simulink model "FCSMPC_new"  (R2026a)
settings: Solver=FixedStepDiscrete  StopTime=inf  FixedStep=SimulinkTs
PreLoadFcn:
  | % Verzeichnis des Modells zum MATLAB-Pfad hinzufügen
  | modelDir = fileparts(get_param(bdroot, 'FileName'));
  | addpath(modelDir);
  | 
  | % Nur der Dateiname – kein Pfad!
  | set_param(bdroot, 'DataDictionary', 'FOC_params.sldd');
model workspace (MAT data in the model file):
  Np : Simulink.Parameter (value not decoded)
undefined symbols (not defined in the file or in its folder): dspblkCoreblockFVToolHelper, FCS, Filter, FOC, FOC_Control_Current_KIid, FOC_Control_Current_KIiq, FOC_Control_Current_KPid, FOC_Control_Current_KPiq, FOC_Control_Current_Krd, FOC_Control_Current_Krq, FOC_Control_Current_TclCur, FOC_Control_Current_Tnd, FOC_Control_Current_Tnq, FOC_Control_InverterVdc_V, FOC_Control_MotorImax_A, FOC_Control_MTPA_MTPV_nT_id_grid, FOC_Control_MTPA_MTPV_nT_iq_grid, FOC_Control_MTPA_MTPV_T_vec, FOC_Control_MTPA_MTPV_w_vec, FOC_Control_OpenLoop_Id_Ref_A, FOC_Control_OpenLoop_Iq_Ref_A, FOC_Control_OpenLoop_Ud_OpenLoop_V, FOC_Control_OpenLoop_Uq_OpenLoop_V, FOC_Control_RF_omegamech_rad_s, FOC_Control_RF_RateCurrent_A, FOC_Control_RF_RateTrq_Nm, FOC_Control_theta_mechOffsetFix, FOC_Control_theta_mechOffsetTime, FOC_Control_TorqueRef_Nm, FOC_Control_Umax_V, FOC_Flag_ClosedLoopControl, FOC_Flag_ControlStrategy, FOC_Flag_PWMEnable, FOC_Flag_ResetControl, FOC_Flag_TorqueControl, FOC_LUT_DQLimiter_DQ_LUTScaling, FOC_PWM_AZSPWMMethod, FOC_PWM_HybridMode, FOC_PWM_LB1, FOC_PWM_LB2, FOC_PWM_PWMManuel, FOC_PWM_RSPWMMethod, FOC_PWM_UB1, FOC_PWM_UB2, FOC_SampleTime_TsCur, gcbh, Plant, SimulinkTs
libraries: hdlsllib x2, autolibfluxpmsm x1, simulink x1
(part 2 of 2)

== matlab function FCSMPC_new/FCS_MPC/SDA_Solve/SDA Solve/Assembly_QP ==
  data: Ad input; Bd input; fd input; H output size=[3*Np 3*Np]; Gamma input; U_unc output size=[3*Np 1]; Phi input; Apow input; Lambdafsw_Ssquare input; Lambdafsw_SE input; Bs_TI input; Iabc input; idiq_ref input; Sin_Cos_Theta input size=[2 1]; Sin_Cos_Theta_Delayed input; wel input; Ts input; U_applied input; regularization input; controllerDelay input; iabcPredictedPrevious input; predictionValid input; iabcCompensated output; deltaIabcBase output; deltaIabcSwitch output; predictionError output size=[3 1]; e_dq output size=[2 1]
function [H, U_unc, iabcCompensated, ...
    deltaIabcBase, deltaIabcSwitch, predictionError, e_dq] = ...
    Assembly_QP(Ad, Bd, fd, Gamma, Phi, Apow, ...
    Lambdafsw_Ssquare, Lambdafsw_SE, Bs_TI, ...
    Iabc, idiq_ref, Sin_Cos_Theta, Sin_Cos_Theta_Delayed, ...
    wel, Ts, U_applied, ...
    regularization, controllerDelay, ...
    iabcPredictedPrevious, predictionValid)
%ASSEMBLY_QP Independent QP-assembly MATLAB Function module.
% Sin_Cos_Theta = [sin(theta_el); cos(theta_el)] at the current instant.
% Sin_Cos_Theta_Delayed is the same signal delayed by one SDA period.
% U_applied is a fixed 6x1 vector delayed by one SDA period and contains the
% two switching vectors that were physically applied during the measurement
% delay, ordered oldest first:
%   U_applied = [Uapply(k-1); UapplySecond(k-1)].
% The last applied switching state is therefore U_applied(4:6).
% With controllerDelay = 40 us and Ts = 20 us, both history steps are used
% to propagate the delayed current measurement to the current instant.
% iabcPredictedPrevious is supplied by a model-level Unit Delay block.

Np = 5;
ns = 3;
nS = ns*Np;

% The surrounding FOC model may provide fixed-point fi signals. This QP
% stage uses matrix factorizations and linear solves, so perform all of its
% numerical work consistently in double precision. Mixing a run-time fi
% value with a non-fi matrix in mtimes is not supported by MATLAB Coder.
Ad = double(Ad);
Bd = double(Bd);
fd = double(fd);
Gamma = double(Gamma);
Phi = double(Phi);
Apow = double(Apow);
Lambdafsw_Ssquare = double(Lambdafsw_Ssquare);
Lambdafsw_SE = double(Lambdafsw_SE);
Bs_TI = double(Bs_TI);
Iabc = double(Iabc);
idiq_ref = double(idiq_ref);
Sin_Cos_Theta = double(Sin_Cos_Theta);
Sin_Cos_Theta_Delayed = double(Sin_Cos_Theta_Delayed);
wel = double(wel);
Ts = double(Ts);
U_applied = double(U_applied);
regularization = double(regularization);
controllerDelay = double(controllerDelay);
iabcPredictedPrevious = double(iabcPredictedPrevious);

sinTheta = Sin_Cos_Theta(1);
cosTheta = Sin_Cos_Theta(2);
thetaCurrent = atan2(sinTheta,cosTheta);
thetaDelayed = atan2( ...
    Sin_Cos_Theta_Delayed(1),Sin_Cos_Theta_Delayed(2));
Talpha_beta = [2/3, -1/3, -1/3; ...
               0, 1/sqrt(3), -1/sqrt(3)];

uprev = U_applied(4:6);

% Reconstruct the present current from the delayed measurement by replaying
% the switching vectors that were physically applied during that delay.
% The fixed upper loop bound keeps dimensions/code generation deterministic.
delaySteps = 0;
if predictionValid
    delaySteps = min(2,max(0,round(controllerDelay/Ts)));
end
iabcCompensated = Iabc;
thetaHistoryStart = thetaCurrent;
if delaySteps == 2
    % The supplied delayed angle is one complete SDA period (2*Ts) old.
    thetaHistoryStart = thetaDelayed;
elseif delaySteps == 1
    % A one-step delay corresponds to the second half of the previous SDA
    % period. The supplied delayed angle is 2*Ts old, so use the current
    % angle and constant-speed assumption to obtain the angle Ts ago.
    thetaHistoryStart = thetaCurrent-wel*Ts;
end
for historyStep = 1:2
    if historyStep <= delaySteps
        thetaHistory = thetaHistoryStart+(historyStep-1)*wel*Ts;
        [deltaBaseHistory,deltaSwitchHistory] = abc_current_increment( ...
            iabcCompensated,thetaHistory,Ad,Bd,fd,Bs_TI,wel,Ts);
        % For two delay steps replay [U1(k-1), U2(k-1)]. For one delay
        % step replay only the most recently applied U2(k-1).
        historySlot = 2-delaySteps+historyStep;
        historyIndices = (historySlot-1)*ns+(1:ns);
        sHistory = U_applied(historyIndices);
        iabcCompensated = iabcCompensated+ ...
            deltaBaseHistory+deltaSwitchHistory*sHistory;
    end
end

% Build the optimization and future-prediction model from the reconstructed
% current state at the current electrical angle.
[deltaIabcBase,deltaIabcSwitch,idiq_fb,Rpark,Bs] = ...
    abc_current_increment( ...
        iabcCompensated,thetaCurrent,Ad,Bd,fd,Bs_TI,wel,Ts);

Upsilon = zeros(2*Np,ns*Np);
for row = 1:Np
    rows = (row-1)*2 + (1:2);
    for col = 1:row
        cols = (col-1)*ns + (1:ns);
        Upsilon(rows,cols) = ...
            Apow((row-col)*2 + (1:2),:)*Bd*Bs;
    end
end

if predictionValid
    predictionError = iabcCompensated-iabcPredictedPrevious;
else
    predictionError = zeros(3,1);
end
e_dq = Rpark*(Talpha_beta*predictionError);

Yref = repmat(idiq_ref,Np,1);
r = Yref-Gamma*idiq_fb-Phi;
W = Upsilon.'*Upsilon + Lambdafsw_Ssquare;
Theta = -Upsilon.'*r-Lambdafsw_SE*uprev;
W = 0.5*(W+W.');
scaleH = max(1,norm(W,'fro'));
W = W+regularization*scaleH*eye(nS);
U_unc = W\(-Theta);

Jx = fliplr(eye(nS));
[Rt,cholFlag] = chol(Jx*W*Jx);
if cholFlag ~= 0
    error('H is not positive definite. Increase lambda_sw or regularization.');
end
H = Jx*Rt*Jx;
end

function [deltaBase,deltaSwitch,idiqState,Rpark,Bs] = ...
    abc_current_increment( ...
        iabcState,thetaEl,Ad,Bd,fd,Bs_TI,wel,Ts)
% One discrete PMSM current step in abc coordinates at thetaEl.
cosTheta = cos(thetaEl);
sinTheta = sin(thetaEl);
Rpark = [cosTheta, sinTheta; -sinTheta, cosTheta];
Talpha_beta = [2/3, -1/3, -1/3; ...
               0, 1/sqrt(3), -1/sqrt(3)];
TinvClarke = [1.0, 0.0; ...
             -0.5, sqrt(3)/2; ...
             -0.5, -sqrt(3)/2];
Jrot = [0 -1; 1 0];

idiqState = Rpark*(Talpha_beta*iabcState);
Bs = Rpark*Bs_TI;
Tdq2abc = TinvClarke*Rpark.';
deltaIdqBase = (Ad-eye(2))*idiqState+fd;
deltaBase = Tdq2abc* ...
    (deltaIdqBase+Jrot*idiqState*(wel*Ts));
deltaSwitch = Tdq2abc*Bd*Bs;
end

== matlab function FCSMPC_new/FCS_MPC/SDA_Solve/SDA Solve/SDA_Solve ==
  data: Jopt output size=[1 1]; nodes output size=[1 1]; optimal output size=[1 1]; H input size=[15 15]; U_unc input size=[15 1]; NmaxNod input size=[1 1]; Uopt output size=[3*Np 1]; Uapply output size=[3]; UoptPrev input size=[15 1]; iabcCompensated input size=[3 1]; deltaIabcBase input size=[3 1]; deltaIabcSwitch input size=[3 3]; lambdaZero input size=[1 1]; lambdaDeadtime input size=[1 1]; deadtime_ratio input size=[1 1]; currentEpsMargin input size=[1 1]; UapplySecond output size=[3 1]; leafNodes output size=[1 1]; bestCMVCost output size=[1 1]; cmvMetricRatio output size=[1 1]; switchCountApplied output size=[1 1]; debug_lower output size=[3 1]; debug_upper output size=[3 1]; iabcPredictedNext output size=[3 1]; Jround output size=[1 1]; Jshift output size=[1 1]; predictionValidNext output boolean size=[1 1]
function [Jopt, nodes, optimal, Uopt, Uapply, UapplySecond, ...
    leafNodes, bestCMVCost, cmvMetricRatio, switchCountApplied, ...
    debug_lower, debug_upper, iabcPredictedNext, ...
    Jround, Jshift, predictionValidNext] = ...
    SDA_Solve(H, U_unc, NmaxNod, UoptPrev, ...
    iabcCompensated, deltaIabcBase, deltaIabcSwitch, ...
    lambdaZero, lambdaDeadtime, deadtime_ratio, currentEpsMargin)
%SDA_SOLVE Independent double-vector SDA MATLAB Function module.
% The first five ports follow FCSMPC_IdealSDA. Feed Uopt back to UoptPrev
% through a Unit Delay initialized with zeros(15,1). Uapply and
% UapplySecond are applied successively for half an external period each.

Np = 5;
ns = 3;
nS = ns*Np;

z = H*U_unc;
s_prev = UoptPrev(4:6);
deadtimeRatio = deadtime_ratio;

Uround = min(max(round(U_unc),0.0),1.0);
Ushift = zeros(nS,1);
Ushift(1:nS-ns) = UoptPrev(ns+1:nS);
Ushift(nS-ns+1:nS) = UoptPrev(nS-ns+1:nS);
Jround = norm(H*(Uround-U_unc),2)^2;
Jshift = norm(H*(Ushift-U_unc),2)^2;
if Jshift < Jround
    U_ini = Ushift;
else
    U_ini = Uround;
end

bestCMVCost = sequence_cmv_cost_predicted( ...
    U_ini,s_prev,iabcCompensated,Np,ns, ...
    deltaIabcBase,deltaIabcSwitch,lambdaZero,lambdaDeadtime, ...
    deadtimeRatio,currentEpsMargin);
bestMetric = norm(H*(U_ini-U_unc),2)^2+bestCMVCost;
bestU = U_ini;

Uwork = zeros(nS,1);
candidatePosition = ones(nS,1);
metricStack = zeros(nS+1,1);
cmvMetricStack = zeros(nS+1,1);
iabcPrediction = zeros(3,Np+1);
iabcPrediction(:,1) = iabcCompensated;
nodes = 0;
leafNodes = 0;
optimal = true;
i = 1;

while i >= 1
    if candidatePosition(i) > 2
        candidatePosition(i) = 1;
        i = i-1;
        continue;
    end
    head = 0.0;
    if i > 1
        head = H(i,1:i-1)*Uwork(1:i-1);
    end
    center = (z(i)-head)/H(i,i);
    if center <= 0.5
        firstCandidate = 0.0;
    else
        firstCandidate = 1.0;
    end
    if candidatePosition(i) == 1
        candidate = firstCandidate;
    else
        candidate = 1.0-firstCandidate;
    end
    candidatePosition(i) = candidatePosition(i)+1;
    Uwork(i) = candidate;
    nodes = nodes+1;
    if NmaxNod > 0 && nodes > NmaxNod
        optimal = false;
        break;
    end

    residual = z(i)-head-H(i,i)*candidate;
    metricNew = metricStack(i)+residual*residual;
    cmvMetricNew = cmvMetricStack(i);
    if mod(i,ns) == 0
        predictionStep = i/ns;
        blockStart = i-ns+1;
        sCurrent = Uwork(blockStart:i);
        if predictionStep == 1
            sPrevious = s_prev;
        else
            sPrevious = Uwork(blockStart-ns:blockStart-1);
        end
        iabcBeforeSwitch = iabcPrediction(:,predictionStep);
        [deltaStep,deltaDead] = deadtime_corrected_current_step( ...
            sPrevious,sCurrent,iabcBeforeSwitch, ...
            deltaIabcBase,deltaIabcSwitch,deadtimeRatio,currentEpsMargin);
        cmvIncrement = cmv_cost( ...
            sPrevious,sCurrent,iabcBeforeSwitch,deltaDead, ...
            lambdaZero,lambdaDeadtime,currentEpsMargin);
        metricNew = metricNew+cmvIncrement;
        cmvMetricNew = cmvMetricNew+cmvIncrement;
        iabcPrediction(:,predictionStep+1) = iabcBeforeSwitch+deltaStep;
    end
    if metricNew > bestMetric
        continue;
    end
    if i == nS
        leafNodes = leafNodes+1;
        if metricNew < bestMetric
            bestMetric = metricNew;
            bestU = Uwork;
            bestCMVCost = cmvMetricNew;
        end
    else
        metricStack(i+1) = metricNew;
        cmvMetricStack(i+1) = cmvMetricNew;
        i = i+1;
        candidatePosition(i) = 1;
    end
end

if isfinite(bestMetric)
    Uopt = bestU;
else
    Uopt = repmat(s_prev,Np,1);
end
Uapply = Uopt(1:3);
UapplySecond = Uopt(4:6);

[deltaFirst,~] = deadtime_corrected_current_step( ...
    s_prev,Uapply,iabcCompensated, ...
    deltaIabcBase,deltaIabcSwitch, ...
    deadtimeRatio,currentEpsMargin);
iabcAfterFirst = iabcCompensated + deltaFirst;

[deltaSecond,~] = deadtime_corrected_current_step( ...
    Uapply,UapplySecond,iabcAfterFirst, ...
    deltaIabcBase,deltaIabcSwitch,deadtimeRatio,currentEpsMargin);
iabcPredictedNext = iabcAfterFirst+deltaSecond;

switchCountApplied = sum(abs(Uapply-s_prev))+ ...
    sum(abs(UapplySecond-Uapply));
Jopt = bestMetric;
if Jopt > eps
    cmvMetricRatio = bestCMVCost/Jopt;
else
    cmvMetricRatio = 0.0;
end
[~,debugDeltaDead] = deadtime_corrected_current_step( ...
    s_prev,Uapply,iabcCompensated,deltaIabcBase,deltaIabcSwitch, ...
    deadtimeRatio,currentEpsMargin);
[~,debug_lower,debug_upper] = cmv_cost( ...
    s_prev,Uapply,iabcCompensated,debugDeltaDead, ...
    lambdaZero,lambdaDeadtime,currentEpsMargin);
predictionValidNext = true;
end

function [deltaStep,deltaDead] = deadtime_corrected_current_step( ...
    sPrevious,sCurrent,iabcBeforeSwitch, ...
    deltaBase,deltaSwitch,deadtimeRatio,currentEps)
sDead = sCurrent;
changed = (sPrevious ~= sCurrent);
signEps = 0.1*currentEps;
for phase = 1:3
    if ~changed(phase)
        continue;
    end
    iPhase = iabcBeforeSwitch(phase);
    if iPhase >= signEps
        sDead(phase) = 0.0;
    elseif iPhase <= -signEps
        sDead(phase) = 1.0;
    else
        sDead(phase) = 0.5*(1.0-iPhase/signEps);
    end
end
sEffective = deadtimeRatio*sDead+(1.0-deadtimeRatio)*sCurrent;
deltaDead = deadtimeRatio*(deltaBase+deltaSwitch*sDead);
deltaStep = deltaBase+deltaSwitch*sEffective;
end

function [penalty,lowerBound,upperBound] = cmv_cost( ...
    sPrevious,sCurrent,iabcBeforeSwitch,deltaDead, ...
    lambdaZero,lambdaDeadtime,currentEpsMargin)
penalty = 0.0;
iabcDeadEnd = iabcBeforeSwitch+deltaDead;
lowerBound = min(iabcBeforeSwitch,iabcDeadEnd)-currentEpsMargin;
upperBound = max(iabcBeforeSwitch,iabcDeadEnd)+currentEpsMargin;
uncertain = (lowerBound <= 0.0) & (upperBound >= 0.0);
if all(sCurrent == 0.0) || all(sCurrent == 1.0)
    penalty = penalty+lambdaZero;
end
changed = (sPrevious ~= sCurrent);
if sum(changed) ~= 2
    return;
end
canBeZero = false(3,1);
canBeOne = false(3,1);
for phase = 1:3
    if ~changed(phase)
        canBeZero(phase) = (sPrevious(phase) == 0.0);
        canBeOne(phase) = (sPrevious(phase) == 1.0);
    elseif uncertain(phase)
        canBeZero(phase) = true;
        canBeOne(phase) = true;
    elseif iabcDeadEnd(phase) > 0.0
        canBeZero(phase) = true;
    else
        canBeOne(phase) = true;
    end
end
if all(canBeZero) || all(canBeOne)
    penalty = penalty+lambdaDeadtime;
end
end

function totalPenalty = sequence_cmv_cost_predicted( ...
    U,s_prev,iabcInitial,Np,ns,deltaBase,deltaSwitch, ...
    lambdaZero,lambdaDeadtime,deadtimeRatio,currentEpsMargin)
totalPenalty = 0.0;
sPrevious = s_prev;
iabcBeforeSwitch = iabcInitial;
for step = 1:Np
    rows = (step-1)*ns+(1:ns);
    sCurrent = U(rows);
    [deltaStep,deltaDead] = deadtime_corrected_current_step( ...
        sPrevious,sCurrent,iabcBeforeSwitch,deltaBase,deltaSwitch, ...
        deadtimeRatio,currentEpsMargin);
    totalPenalty = totalPenalty+cmv_cost( ...
        sPrevious,sCurrent,iabcBeforeSwitch,deltaDead, ...
        lambdaZero,lambdaDeadtime,currentEpsMargin);
    iabcBeforeSwitch = iabcBeforeSwitch+deltaStep;
    sPrevious = sCurrent;
end
end

== stateflow chart FCSMPC_new/FCS_MPC/CurrentRefCalc/Current_RateLimiter/RateLimiter ==
  settings: updateMethod=DISCRETE  sampleTime=FOC.SampleTime.TsSpeed
  state IDLE
  state Rising
    entry:  y =  fi(y_prev +dT * R, 1, 32, 18);
    exit: y_prev = y;
  state Falling
    entry:  y = fi(y_prev+dT * F, 1, 32, 18);
    exit: y_prev = y;
  state Directpassage
    entry:  y = u;
    exit: y_prev = y;
  (default) -> IDLE
  IDLE -> (junction 22)
  (junction 22) -> Rising [order 1] : [(u-y_prev)/dT>=R]
  (junction 22) -> Falling [order 2] : [(u-y_prev)/dT<=F]
  Rising -> (junction 22)
  Falling -> (junction 22)
  Directpassage -> (junction 22)
  (junction 22) -> Directpassage [order 3] : [(u-y_prev)/dT<R && (u-y_prev)/dT>F]
  data: u input fixdt(1,32,18); R input fixdt(1,32,18); F input fixdt(1,32,18); dT constant fixdt(1,32,18) size=1 =FOC.SampleTime.TsSpeed; y output fixdt(1,32,18); y_prev local fixdt(1,32,18) =0

== stateflow chart FCSMPC_new/FCS_MPC/CurrentRefCalc/Current_RateLimiter/RateLimiter1 ==
  settings: updateMethod=DISCRETE  sampleTime=FOC.SampleTime.TsSpeed
  state IDLE
  state Rising
    entry:  y =  fi(y_prev +dT * R, 1, 32, 18);
    exit: y_prev = y;
  state Falling
    entry:  y = fi(y_prev+dT * F, 1, 32, 18);
    exit: y_prev = y;
  state Directpassage
    entry:  y = u;
    exit: y_prev = y;
  (default) -> IDLE
  IDLE -> (junction 22)
  (junction 22) -> Rising [order 1] : [(u-y_prev)/dT>=R]
  (junction 22) -> Falling [order 2] : [(u-y_prev)/dT<=F]
  Rising -> (junction 22)
  Falling -> (junction 22)
  Directpassage -> (junction 22)
  (junction 22) -> Directpassage [order 3] : [(u-y_prev)/dT<R && (u-y_prev)/dT>F]
  data: u input fixdt(1,32,18); R input fixdt(1,32,18); F input fixdt(1,32,18); dT constant fixdt(1,32,18) size=1 =FOC.SampleTime.TsSpeed; y output fixdt(1,32,18); y_prev local fixdt(1,32,18) =0

== stateflow chart FCSMPC_new/FCS_MPC/CurrentRefCalc/RateLimiter ==
  settings: updateMethod=DISCRETE  sampleTime=FOC.SampleTime.TsSpeed
  state IDLE
  state Rising
    entry:  y =  fi(y_prev +dT * R, 1, 32, 18);
    exit: y_prev = y;
  state Falling
    entry:  y = fi(y_prev+dT * F, 1, 32, 18);
    exit: y_prev = y;
  state Directpassage
    entry:  y = u;
    exit: y_prev = y;
  (default) -> IDLE
  IDLE -> (junction 22)
  (junction 22) -> Rising [order 1] : [(u-y_prev)/dT>=R]
  (junction 22) -> Falling [order 2] : [(u-y_prev)/dT<=F]
  Rising -> (junction 22)
  Falling -> (junction 22)
  Directpassage -> (junction 22)
  (junction 22) -> Directpassage [order 3] : [(u-y_prev)/dT<R && (u-y_prev)/dT>F]
  data: u input fixdt(1,32,18); R input fixdt(1,32,18); F input fixdt(1,32,18); dT constant fixdt(1,32,18) size=1 =FOC.SampleTime.TsSpeed; y output fixdt(1,32,18); y_prev local fixdt(1,32,18) =0
